simulink model "PID_correection_hardware"  (R2025a)
settings: Solver=FixedStepDiscrete  StartTime=0.0  StopTime=inf  FixedStep=Ts  RelTol=1e-3  EnableMultiTasking=on
InitFcn:
  | addpath('functions');
model workspace (MATLAB code in the model file):
  | arm_torque = 0;
  | L_arm = 0.115;
  | I_arm = 6.5e-4;
  | lcom_1 = 0.058;
  | I_1 = 3.7e-5;
  | m_1 = 0.023;
  | L_1 = 0.13;
  | Ts = 0.0001
  | 
  | init_cond = [pi/2; 0; 0.26; 0];
libraries: simulink x3, stm32f4xxblockslib x3, slpidlib x2, stm32blockslib x2
settings Model: STM32="{\"AnalogInput\":{\"ID\":\"PID_correection_ideal_parametertest:153\"},\"PWMOutput\":[{\"ID\":\"PID_correection_ideal_parametertest:154\"},{\"ID\":\"PID_correection_hardware:172\"}],\"DigitalPortRead\":{\"ID\":\"PID_correection_ideal_parametertest:155\"},\"EncoderBlock\":[{\"ID\":\"PID_correection_ideal_parametertest:156\"},{\"ID\":\"PID_correection_hardware:156\"},{\"ID\":\"PID_correection_hardware:167\"}],\"I2CControllerRead\":{\"ID\":\"PID_correection_ideal_parametertest:158\"},\"DigitalPortWrite\":[{\"ID\":\"PID_correection_hardware:178\"},{\"ID\":\"PID_correection_hardware:179\"}]}"  PacingRate=0.400000  Creator=Esther  LastModifiedBy=NKW
settings SolverCC: AutoInsertRateTranBlk=on
settings OptimizationCC: DefaultParameterBehavior=Inlined  EnhancedBackFolding=on  PassReuseOutputArgsAs=Individual arguments  ZeroExternalMemoryAtStartup=off  ZeroInternalMemoryAtStartup=off  MaxStackSize=512  OptimizeBlockOrder=speed  DifferentSizesBufferReuse=on  OptimizationCustomize=off  EfficientTunableParamExpr=on
settings DebuggingCC: ParameterTunabilityLossMsg=error
settings HardwareCC: ProdBitPerPointer=32.0  ProdBitPerSizeT=32.0  ProdBitPerPtrDiffT=32.0  ProdLargestAtomicInteger=Long  ProdLargestAtomicFloat=Double  ProdWordSize=32.0  ProdLongLongMode=on  ProdHWDeviceType=ARM Compatible->ARM Cortex-M
settings RTWCC: SystemTargetFile=ert.tlc  HardwareBoard=STM32F4xx Based  TemplateMakefile=ert_default_tmf  Toolchain=Armclang Compiler  Description=Embedded Coder
settings CodeAppCC: ForceParamTrailComments=on  IgnoreCustomStorageClasses=off  OperatorAnnotations=on  SimulinkDataObjDesc=on  SFDataObjDesc=on  InsertBlockDesc=on
settings ERTTargetCC: ExtModeTransport=3.0  ExtModeStaticAllocSize=2048.0  TargetLangStandard=C99 (ISO)  CodeReplacementLibrary=ARM Cortex-M

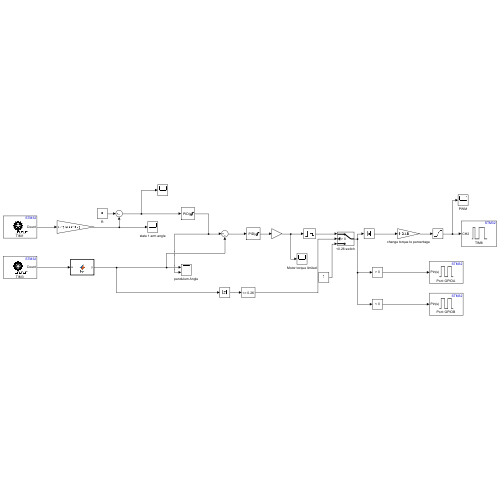
[thumbnail: Simulink's stored preview of the top-level diagram]
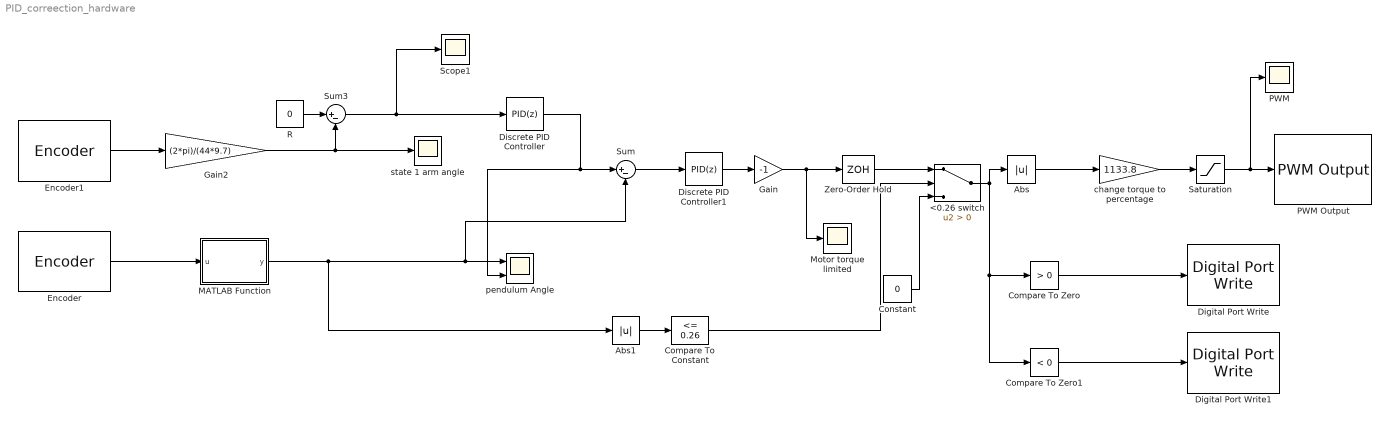
== system PID_correection_hardware ==
  <0.26 switch : Switch  Criteria=u2 > Threshold  SaturateOnIntegerOverflow=off  InputSameDT=off
  Abs : Abs  SaturateOnIntegerOverflow=off
  Abs1 : Abs  SaturateOnIntegerOverflow=off
  Compare To Constant : simulink/Logic and Bit Operations/Compare To Constant  relop=<=  const=0.26  OutDataTypeStr=uint8
  Compare To Zero : simulink/Logic and Bit Operations/Compare To Zero  relop=>  OutDataTypeStr=uint8
  Compare To Zero1 : simulink/Logic and Bit Operations/Compare To Zero  relop=<  OutDataTypeStr=uint8
  Constant : Constant  Value=0
  Digital Port Write : stm32f4xxblockslib/Digital Port Write  PortName=GPIOA  PinNumber=[10]  ReadOperation=off  IOAsArray=on  EnableSimPort=off  hoistedMaskSrc=ECSoC/ECSimCodegen/Digital Port Write
  Digital Port Write1 : stm32f4xxblockslib/Digital Port Write  PortName=GPIOB  PinNumber=[3]  ReadOperation=off  IOAsArray=on  EnableSimPort=off  hoistedMaskSrc=ECSoC/ECSimCodegen/Digital Port Write
  Discrete PID Controller : slpidlib/PID Controller  Controller=PID  Form=Parallel  TimeDomain=Discrete-time  UseExternalTs=off  SampleTime=Ts  IntegratorMethod=Forward Euler  FilterMethod=Forward Euler  ControllerParametersSource=internal  P=0.05  I=0  UseKiTs=on  D=0.08  UseExternalDerivativeSource=off  N=8  UseFilter=on  TunerSelectOption=Transfer Function Based (PID Tuner App)  InitialConditionSource=internal  InitialConditionForIntegrator=0  InitialConditionForFilter=0  DifferentiatorICPrevScaledInput=0  ExternalReset=none  TrackingMode=off  Kt=1  LimitOutput=on  SatLimitsSource=internal  UpperSaturationLimit=0.1  LowerSaturationLimit=-0.1  LinearizeAsGain=off  AntiWindupMode=none  Kb=1  LimitIntegrator=off  UpperIntegratorSaturationLimit=inf  LowerIntegratorSaturationLimit=-inf  POutMin=[]  POutMax=[]  IOutMin=[]  IOutMax=[]  DOutMin=[]  DOutMax=[]  NOutMin=[]  NOutMax=[]  SumOutMin=[]  SumOutMax=[]  SaturationOutMin=[]  SaturationOutMax=[]  PParamMin=[]  PParamMax=[]  IParamMin=[]  IParamMax=[]  DParamMin=[]  DParamMax=[]  NParamMin=[]  NParamMax=[]  KbParamMin=[]  KbParamMax=[]  KtParamMin=[]  KtParamMax=[]  KbOutMin=[]  KbOutMax=[]  KtOutMin=[]  KtOutMax=[]  IntegratorOutMin=[]  IntegratorOutMax=[]  FilterOutMin=[]  FilterOutMax=[]  SumI1OutMin=[]  SumI1OutMax=[]  SumI2OutMin=[]  SumI2OutMax=[]  SumI3OutMin=[]  SumI3OutMax=[]  SumI4OutMin=[]  SumI4OutMax=[]  SumDOutMin=[]  SumDOutMax=[]  DifferentiatorOutMin=[]  DifferentiatorOutMax=[]  FilterDiffOutCoefMin=[]  FilterDiffOutCoefMax=[]  ReciprocalOutMin=[]  ReciprocalOutMax=[]  SumDenOutMin=[]  SumDenOutMax=[]  SumNumOutMin=[]  SumNumOutMax=[]  DivideOutMin=[]  DivideOutMax=[]  UdiffTsProdOutMin=[]  UdiffTsProdOutMax=[]  NTsProdOutMin=[]  NTsProdOutMax=[]  UintegralTsProdOutMin=[]  UintegralTsProdOutMax=[]  UngainTsProdOutMin=[]  UngainTsProdOutMax=[]  ClampingZeroOutDataTypeStr=Inherit: Inherit via back propagation  ClampingZeroOutMin=[]  ClampingZeroOutMax=[]  FilterDenConstantOutDataTypeStr=Inherit: Inherit via back propagation  FilterDenConstantOutMin=[]  FilterDenConstantOutMax=[]  PCopyOutDataTypeStr=Inherit: Inherit via back propagation  PCopyOutMin=[]  PCopyOutMax=[]  NCopyOutDataTypeStr=Inherit: Inherit via back propagation  NCopyOutMin=[]  NCopyOutMax=[]  IntegratorContinuousStateAttributes=''  IntegratorStateMustResolveToSignalObject=off  IntegratorRTWStateStorageClass=Auto  FilterContinuousStateAttributes=''  FilterStateMustResolveToSignalObject=off  FilterRTWStateStorageClass=Auto  ParallelPVariant=InternalParameters  IdealPVariant=Disabled  IVariant=InternalParameters  DVariant=InternalParameters  IntegratorVariant=Discrete  SatVariant=Enabled  AWVariant=Passthrough  PCopyVariant=Disabled  TRVariant=Disabled  FdbkBlocksVariant=Forward  IdealPFdbkVariant=Disabled  SatFdbkVariant=Disabled  DerivativeFilterVariant=ForwardEulerFilter  NVariant=InternalParameters  NCopyVariant=Disabled  FilterICVariant=InternalICsFilter  IntegratorICVariant=InternalICs  ExternalResetVariant=Disabled  TRSumVariant=Passthrough  SumFdbkVariant=Disabled  SumVariant=Sum_PID  TsampFilterVariant=InternalTs  TsampNgainVariant=Passthrough  TsampIntegralVariant=Disabled_SignalSpec  ExternalSaturationOutDataTypeStr=Inherit: Same as second input  DerivativeSourceVariant=ErrorSignal  PreIntVariant=InternalPreInt
      settings: LibrarySourceBlock=simulink/Discrete/Discrete PID Controller
  Discrete PID Controller1 : slpidlib/PID Controller  Controller=PID  Form=Parallel  TimeDomain=Discrete-time  UseExternalTs=off  SampleTime=Ts  IntegratorMethod=Forward Euler  FilterMethod=Forward Euler  ControllerParametersSource=internal  P=60  I=0  UseKiTs=on  D=2  UseExternalDerivativeSource=off  N=50  UseFilter=on  TunerSelectOption=Transfer Function Based (PID Tuner App)  InitialConditionSource=internal  InitialConditionForIntegrator=0  InitialConditionForFilter=0  DifferentiatorICPrevScaledInput=0  ExternalReset=none  TrackingMode=off  Kt=1  LimitOutput=on  SatLimitsSource=internal  UpperSaturationLimit=0.088  LowerSaturationLimit=-0.088  LinearizeAsGain=off  AntiWindupMode=clamping  Kb=1  LimitIntegrator=off  UpperIntegratorSaturationLimit=inf  LowerIntegratorSaturationLimit=-inf  POutMin=[]  POutMax=[]  IOutMin=[]  IOutMax=[]  DOutMin=[]  DOutMax=[]  NOutMin=[]  NOutMax=[]  SumOutMin=[]  SumOutMax=[]  SaturationOutMin=[]  SaturationOutMax=[]  PParamMin=[]  PParamMax=[]  IParamMin=[]  IParamMax=[]  DParamMin=[]  DParamMax=[]  NParamMin=[]  NParamMax=[]  KbParamMin=[]  KbParamMax=[]  KtParamMin=[]  KtParamMax=[]  KbOutMin=[]  KbOutMax=[]  KtOutMin=[]  KtOutMax=[]  IntegratorOutMin=[]  IntegratorOutMax=[]  FilterOutMin=[]  FilterOutMax=[]  SumI1OutMin=[]  SumI1OutMax=[]  SumI2OutMin=[]  SumI2OutMax=[]  SumI3OutMin=[]  SumI3OutMax=[]  SumI4OutMin=[]  SumI4OutMax=[]  SumDOutMin=[]  SumDOutMax=[]  DifferentiatorOutMin=[]  DifferentiatorOutMax=[]  FilterDiffOutCoefMin=[]  FilterDiffOutCoefMax=[]  ReciprocalOutMin=[]  ReciprocalOutMax=[]  SumDenOutMin=[]  SumDenOutMax=[]  SumNumOutMin=[]  SumNumOutMax=[]  DivideOutMin=[]  DivideOutMax=[]  UdiffTsProdOutMin=[]  UdiffTsProdOutMax=[]  NTsProdOutMin=[]  NTsProdOutMax=[]  UintegralTsProdOutMin=[]  UintegralTsProdOutMax=[]  UngainTsProdOutMin=[]  UngainTsProdOutMax=[]  ClampingZeroOutDataTypeStr=Inherit: Inherit via back propagation  ClampingZeroOutMin=[]  ClampingZeroOutMax=[]  FilterDenConstantOutDataTypeStr=Inherit: Inherit via back propagation  FilterDenConstantOutMin=[]  FilterDenConstantOutMax=[]  PCopyOutDataTypeStr=Inherit: Inherit via back propagation  PCopyOutMin=[]  PCopyOutMax=[]  NCopyOutDataTypeStr=Inherit: Inherit via back propagation  NCopyOutMin=[]  NCopyOutMax=[]  IntegratorContinuousStateAttributes=''  IntegratorStateMustResolveToSignalObject=off  IntegratorRTWStateStorageClass=Auto  FilterContinuousStateAttributes=''  FilterStateMustResolveToSignalObject=off  FilterRTWStateStorageClass=Auto  ParallelPVariant=InternalParameters  IdealPVariant=Disabled  IVariant=InternalParameters  DVariant=InternalParameters  IntegratorVariant=Discrete  SatVariant=Enabled  AWVariant=DiscClampingParallel  PCopyVariant=Disabled  TRVariant=Disabled  FdbkBlocksVariant=Forward  IdealPFdbkVariant=Disabled  SatFdbkVariant=Disabled  DerivativeFilterVariant=ForwardEulerFilter  NVariant=InternalParameters  NCopyVariant=Disabled  FilterICVariant=InternalICsFilter  IntegratorICVariant=InternalICs  ExternalResetVariant=Disabled  TRSumVariant=Passthrough  SumFdbkVariant=Disabled  SumVariant=Sum_PID  TsampFilterVariant=InternalTs  TsampNgainVariant=Passthrough  TsampIntegralVariant=Disabled_SignalSpec  ExternalSaturationOutDataTypeStr=Inherit: Same as second input  DerivativeSourceVariant=ErrorSignal  PreIntVariant=InternalPreInt
      settings: LibrarySourceBlock=simulink/Discrete/Discrete PID Controller
  Encoder : stm32blockslib/Encoder  TimerModule=TIM3  EnableResetInput=off  OutputDirection=off  SampleTime=Ts
      settings: LibrarySourceBlock=stm32f4xxblockslib/Encoder
  Encoder1 : stm32blockslib/Encoder  TimerModule=TIM1  EnableResetInput=off  OutputDirection=off  SampleTime=Ts
      settings: LibrarySourceBlock=stm32f4xxblockslib/Encoder
  Gain : Gain  Gain=-1
  Gain2 : Gain  Gain=(2*pi)/(44*9.7)
  MATLAB Function : MATLAB Function  TreatAsAtomicUnit=on
  Motor torque limited : Scope
      settings: ActiveDisplayYMinimum=-0.10999999999999999  ActiveDisplayYMaximum=0.10999999999999999  DataLoggingVariableName=ScopeData5
  PWM : Scope
      settings: DataLoggingVariableName=ScopeData2
  PWM Output : stm32f4xxblockslib/PWM Output  ProcessorFamily=STM32F4  TimerModule=TIM8  DutycycleUnits=Percentage  EnableChannel1=off  EnableCaptureCompare1Input=off  EnableCaptureCompare1ComplementaryInput=off  EnableOutputCompare1ModeInput=off  EnableChannel2=on  EnableCaptureCompare2Input=off  EnableCaptureCompare2ComplementaryInput=off  EnableOutputCompare2ModeInput=off  EnableChannel3=off  EnableCaptureCompare3Input=off  EnableCaptureCompare3ComplementaryInput=off  EnableOutputCompare3ModeInput=off  EnableChannel4=off  EnableCaptureCompare4Input=off  EnableCaptureCompare4ComplementaryInput=off  EnableOutputCompare4ModeInput=off  EnableChannel5=off  EnableCaptureCompare5Input=off  EnableOutputCompare5ModeInput=off  EnableChannel6=off  EnableCaptureCompare6Input=off  EnableOutputCompare6ModeInput=off  EnableCounterInput=off  EnableMainOutputInput=off  EnableFrequencyInput=off  SetRCAfterCE=off  OutputDirection=off  OutputMainOutputEnableStatus=off  SampleTime=0.1  EnableSimPort=off  EnableUpdateEvent=off  EnableCaptureCompare1Event=off  EnableCaptureCompare2Event=off  EnableCaptureCompare3Event=off  EnableCaptureCompare4Event=off  EnableTriggerEvent=off  EnableBreakEvent=off  EnableBreakEvent2=off  hoistedMaskSrc=ECSoC/ECSimCodegen/PWM Output
  R : Constant  Value=0
  Saturation : Saturate  UpperLimit=100  LowerLimit=0
  Scope1 : Scope
      settings: ActiveDisplayYMinimum=-1  ActiveDisplayYMaximum=1  DataLoggingVariableName=ScopeData3
  Sum : Sum  Inputs=|+-
  Sum3 : Sum  Inputs=|+-
  Zero-Order Hold : ZeroOrderHold  SampleTime=-1
  change torque to percentage : Gain  Gain=1133.8
  pendulum Angle : Scope  NumInputPorts=2
      settings: ActiveDisplayYMinimum=-0.14582152994796849  ActiveDisplayYMaximum=0.30509128110532979  DataLoggingVariableName=ScopeData6
  state 1 arm angle : Scope
      settings: ActiveDisplayYMinimum=-0.33874782734308273  ActiveDisplayYMaximum=2.8578499042965384
  wires:
  R/1 -> Sum3/1
  Sum3/1 -> Scope1/1, Discrete PID Controller/1
  Gain/1 -> Motor torque limited/1, Zero-Order Hold/1
  Gain2/1 -> Sum3/2, state 1 arm angle/1
  MATLAB Function/1(y) -> Abs1/1, Sum/2, pendulum Angle/1
  Discrete PID Controller/1 -> pendulum Angle/2, Sum/1
  Sum/1 -> Discrete PID Controller1/1
  Discrete PID Controller1/1 -> Gain/1
  Encoder/1 -> MATLAB Function/1(u)
  Encoder1/1 -> Gain2/1
  Compare To Zero/1 -> Digital Port Write/1
  Compare To Zero1/1 -> Digital Port Write1/1
  Abs/1 -> change torque to percentage/1
  change torque to percentage/1 -> Saturation/1
  Saturation/1 -> PWM/1, PWM Output/1
  Zero-Order Hold/1 -> <0.26 switch/1
  Abs1/1 -> Compare To Constant/1
  Compare To Constant/1 -> <0.26 switch/2
  Constant/1 -> <0.26 switch/3
  <0.26 switch/1 -> Abs/1, Compare To Zero1/1, Compare To Zero/1

== matlab function PID_correection_hardware/MATLAB Function ==
  data: u input; y output
function y = fcn(u)
    % 此时 u 是 TIM3 输出的原始脉冲数 (int32)
    u_single = single(u);
    
    % 在函数内部一次性完成：换算 -> 模运算 -> 平移
    deg_accumulated = (u_single / 8000.0) * (2*pi);
    y = mod(deg_accumulated, 2*pi) - pi;
end
